simulink model "H_inf_SIMULINK"  (R2026a)
settings: Solver=VariableStepAuto  StopTime=50
values from neighbouring files (symbols this model uses):
  DIRK = K1    [T1_Hinf_Dir.m]    (also in T1_Hinf_Dir_v2.m)
  LATK = K1    [T1_Hinf_Lat.m]
  linmodel =     [modelo_lin.mat]
undefined symbols (not defined in the file or in its folder): LONK
libraries: simulink x4
settings Model: Creator=sslan  LastModifiedBy=caden

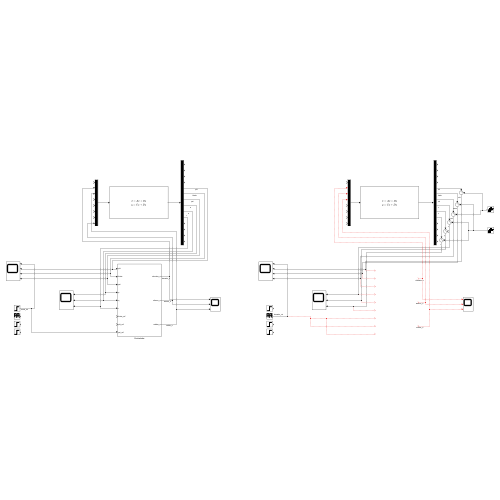
[thumbnail: Simulink's stored preview of the top-level diagram]
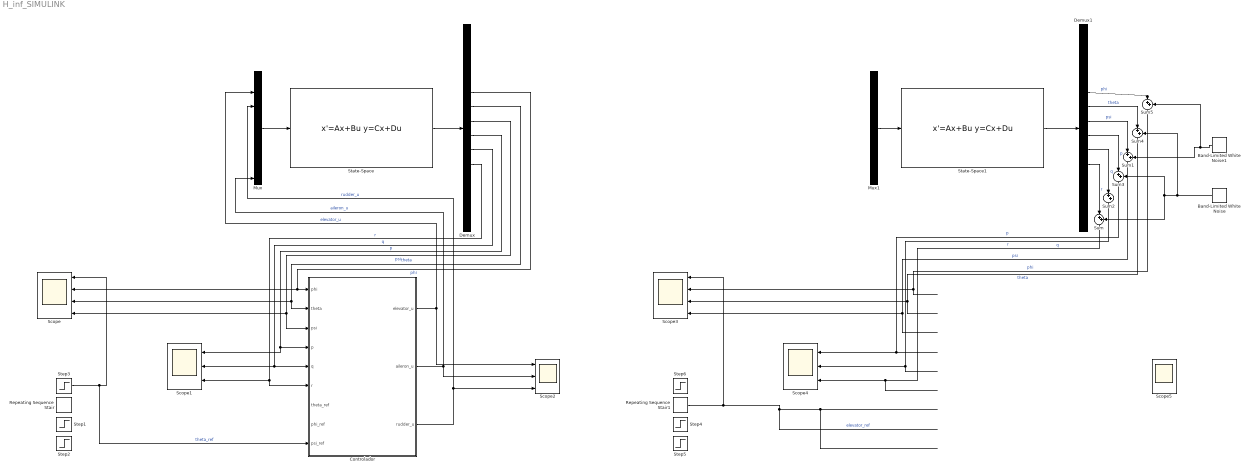
== system H_inf_SIMULINK ==
  Band-Limited White Noise : simulink/Sources/Band-Limited White Noise  Cov=[0.001]  Ts=0.1  seed=[23341]
  Band-Limited White Noise1 : simulink/Sources/Band-Limited White Noise  Cov=[0.0001]  Ts=0.1  seed=[23341]
  Controlador : Subsystem
  Demux : Demux  Outputs=14
  Demux1 : Demux  Outputs=14
  Mux : Mux  Inputs=8
  Mux1 : Mux  Inputs=8
  Repeating Sequence Stair : simulink/Sources/Repeating Sequence Stair  OutValues=[2 2 -2 2 2 -2].'  tsamp=10  OutMin=[]  OutMax=[]  OutDataTypeStr=double  OutputDataTypeScalingMode=double  OutDataType=fixdt(0,8)  ConRadixGroup=Best Precision: Vector-wise  OutScaling=2^-12
  Repeating Sequence Stair1 : simulink/Sources/Repeating Sequence Stair  OutValues=[2 2 -2 2 2 -2].'  tsamp=10  OutMin=[]  OutMax=[]  OutDataTypeStr=double  OutputDataTypeScalingMode=double  OutDataType=fixdt(0,8)  ConRadixGroup=Best Precision: Vector-wise  OutScaling=2^-12
  Scope : Scope  NumInputPorts=4
      settings: ActiveDisplayYMinimum=-50.08001  ActiveDisplayYMaximum=50.30667
  Scope{1..2,4..5} (4 alike) : Scope  NumInputPorts=3
      Scope1 settings: ActiveDisplayYMinimum=-152.7528  ActiveDisplayYMaximum=257.85359
      Scope2 settings: ActiveDisplayYMinimum=-6.0997  ActiveDisplayYMaximum=5.46406  DataLoggingVariableName=ScopeData2
      Scope4 settings: ActiveDisplayYMinimum=-406.19977  ActiveDisplayYMaximum=457.66486  DataLoggingVariableName=ScopeData4
      Scope5 settings: ActiveDisplayYMinimum=-37.5  ActiveDisplayYMaximum=37.5  DataLoggingVariableName=ScopeData5
  Scope3 : Scope  NumInputPorts=4
      settings: ActiveDisplayYMinimum=-13.26649  ActiveDisplayYMaximum=13.38271  DataLoggingVariableName=ScopeData3
  State-Space : StateSpace  A=linmodel.A  B=linmodel.B  C=linmodel.C  D=linmodel.D  InitialCondition=0
  State-Space1 : StateSpace  A=linmodel.A  B=linmodel.B  C=linmodel.C  D=linmodel.D  InitialCondition=0
  Step{1..2,4..5} (4 alike) : Step  FinalValue=40  SampleTime=0
  Step3 : Step  Time=15  InitialValue=-40  FinalValue=40  SampleTime=0
  Step6 : Step  InitialValue=-40  FinalValue=40  SampleTime=0
  Sum{,1..5} (6 alike) : Sum  Inputs=|++
  wires:
  Mux/1 -> State-Space/1
  State-Space/1 -> Demux/1
  Demux/6 -> Controlador/2(theta), Scope/3  "theta"
  Demux/7 -> Controlador/3(psi), Scope/4  "psi"
  Demux/8 -> Scope1/1, Controlador/4(p)  "p"
  Demux/9 -> Controlador/5(q), Scope1/2  "q"
  Demux/10 -> Controlador/6(r), Scope1/3  "r"
  Step3/1 -> Controlador/9(psi_ref), Scope/1  "theta_ref"
  Controlador/1(elevator_u) -> Mux/2, Scope2/1  "elevator_u"
  Controlador/2(aileron_u) -> Mux/8, Scope2/2  "aileron_u"
  Controlador/3(rudder_u) -> Mux/3, Scope2/3  "rudder_u"
  Demux/5 -> Scope/2, Controlador/1(phi)  "phi"
  Repeating Sequence Stair1/1 -> Scope3/1  "elevator_ref"
  ? -> Mux1/3, Scope5/2  "aileron_u"
  Sum/1 -> Scope4/3  "r"
  Sum5/1 -> Scope3/2  "phi"
  ? -> Scope5/3, Mux1/4  "rudder_u"
  Mux1/1 -> State-Space1/1
  ? -> Mux1/2, Scope5/1  "elevator_u"
  State-Space1/1 -> Demux1/1
  Sum2/1 -> Scope4/2  "q"
  Sum4/1 -> Scope3/3  "theta"
  Sum1/1 -> Scope3/4  "psi"
  Sum3/1 -> Scope4/1  "p"
  Demux1/10 -> Sum/1  "r"
  Band-Limited White Noise/1 -> Sum4/2, Sum3/2, Sum/2
  Demux1/9 -> Sum2/1  "q"
  Demux1/8 -> Sum3/1  "p"
  Demux1/7 -> Sum1/1  "psi"
  Demux1/6 -> Sum4/1  "theta"
  Demux1/5 -> Sum5/1  "phi"
  Band-Limited White Noise1/1 -> Sum5/2, Sum1/2

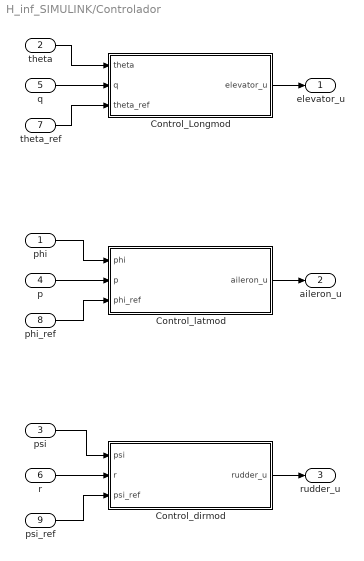
== system H_inf_SIMULINK/Controlador ==
  phi : Inport
  theta : Inport  Port=2
  psi : Inport  Port=3
  p : Inport  Port=4
  q : Inport  Port=5
  r : Inport  Port=6
  theta_ref : Inport  Port=7
  phi_ref : Inport  Port=8
  psi_ref : Inport  Port=9
  Control_Longmod : Subsystem
  Control_dirmod : Subsystem
  "Control_latmod " : Subsystem
  elevator_u : Outport
  aileron_u : Outport  Port=2
  rudder_u : Outport  Port=3
  wires:
  psi_ref/1 -> Control_dirmod/3(psi_ref)
  phi_ref/1 -> "Control_latmod "/3(phi_ref)
  r/1 -> Control_dirmod/2(r)
  p/1 -> "Control_latmod "/2(p)
  theta_ref/1 -> Control_Longmod/3(theta_ref)
  phi/1 -> "Control_latmod "/1(phi)
  theta/1 -> Control_Longmod/1(theta)
  q/1 -> Control_Longmod/2(q)
  Control_Longmod/1(elevator_u) -> elevator_u/1
  psi/1 -> Control_dirmod/1(psi)
  "Control_latmod "/1(aileron_u) -> aileron_u/1
  Control_dirmod/1(rudder_u) -> rudder_u/1

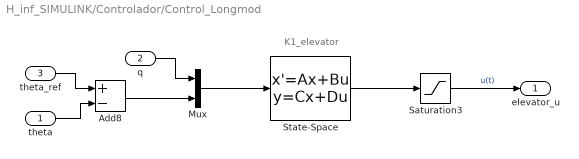
== system H_inf_SIMULINK/Controlador/Control_Longmod ==
  note: K1_elevator
  theta : Inport
  q : Inport  Port=2
  theta_ref : Inport  Port=3
  Add8 : Sum  Inputs=+-
  Mux : Mux  Inputs=2
  Saturation3 : Saturate  UpperLimit=30  LowerLimit=-30
  State-Space : StateSpace  A=LONK.A  B=LONK.B  C=LONK.C  D=LONK.D  InitialCondition=0
  elevator_u : Outport
  wires:
  Saturation3/1 -> elevator_u/1  "u(t)"
  State-Space/1 -> Saturation3/1
  Add8/1 -> Mux/2
  q/1 -> Mux/1
  theta_ref/1 -> Add8/1
  theta/1 -> Add8/2
  Mux/1 -> State-Space/1

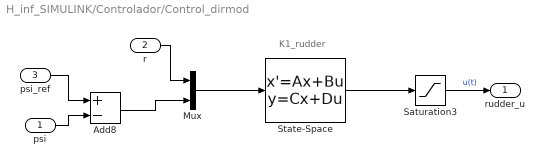
== system H_inf_SIMULINK/Controlador/Control_dirmod ==
  note: K1_rudder
  psi : Inport
  r : Inport  Port=2
  psi_ref : Inport  Port=3
  Add8 : Sum  Inputs=+-
  Mux : Mux  Inputs=2
  Saturation3 : Saturate  UpperLimit=30  LowerLimit=-30
  State-Space : StateSpace  A=DIRK.A  B=DIRK.B  C=DIRK.C  D=DIRK.D  InitialCondition=0
  rudder_u : Outport
  wires:
  psi_ref/1 -> Add8/1
  Saturation3/1 -> rudder_u/1  "u(t)"
  psi/1 -> Add8/2
  State-Space/1 -> Saturation3/1
  Mux/1 -> State-Space/1
  r/1 -> Mux/1
  Add8/1 -> Mux/2

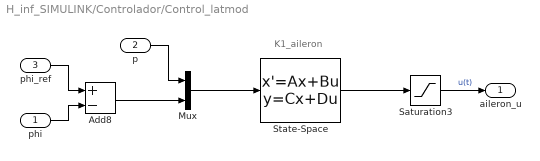
== system H_inf_SIMULINK/Controlador/Control_latmod  ==
  note: K1_aileron
  phi : Inport
  p : Inport  Port=2
  phi_ref : Inport  Port=3
  Add8 : Sum  Inputs=+-
  Mux : Mux  Inputs=2
  Saturation3 : Saturate  UpperLimit=30  LowerLimit=-30
  State-Space : StateSpace  A=LATK.A  B=LATK.B  C=LATK.C  D=LATK.D  InitialCondition=0
  aileron_u : Outport
  wires:
  phi_ref/1 -> Add8/1
  Saturation3/1 -> aileron_u/1  "u(t)"
  Add8/1 -> Mux/2
  phi/1 -> Add8/2
  State-Space/1 -> Saturation3/1
  p/1 -> Mux/1
  Mux/1 -> State-Space/1
